simulink model "DAB_Converter_CPPS"  (R2025b)
settings: Solver=VariableStepAuto  StartTime=0.0  StopTime=inf  FixedStep=0.01  RelTol=1e-3
InitFcn:
  | % % 예시 코드 (SCPI 통신 객체가 obj_psu 라고 가정)
  | % % 시뮬레이션 시작 전에 미리 40V를 쏴줍니다.
  | % fprintf(obj_psu, 'VOLT 40');
  | % pause(0.5); % 장비가 인식할 시간 0.5초 대기
  | % disp('Initial Voltage Set to 40V');
undefined symbols (not defined in the file): dspblkCoreblockFVToolHelper, gcbh
libraries: instrumentseriallib x3, simulink x1, sldrtlib x1
settings Model: DataDictionary=DAB_Parameters.sldd  Creator=JWS  LastModifiedBy=pys30
settings DataIOCC: LimitDataPoints=on  MaxDataPoints=10000  SignalLogging=off  DSMLogging=off  ReturnWorkspaceOutputs=off

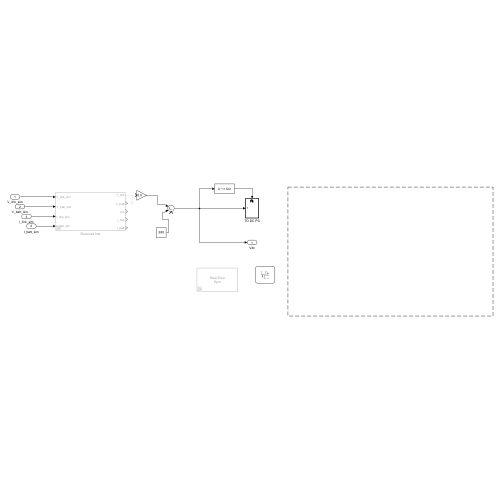
[thumbnail: Simulink's stored preview of the top-level diagram]
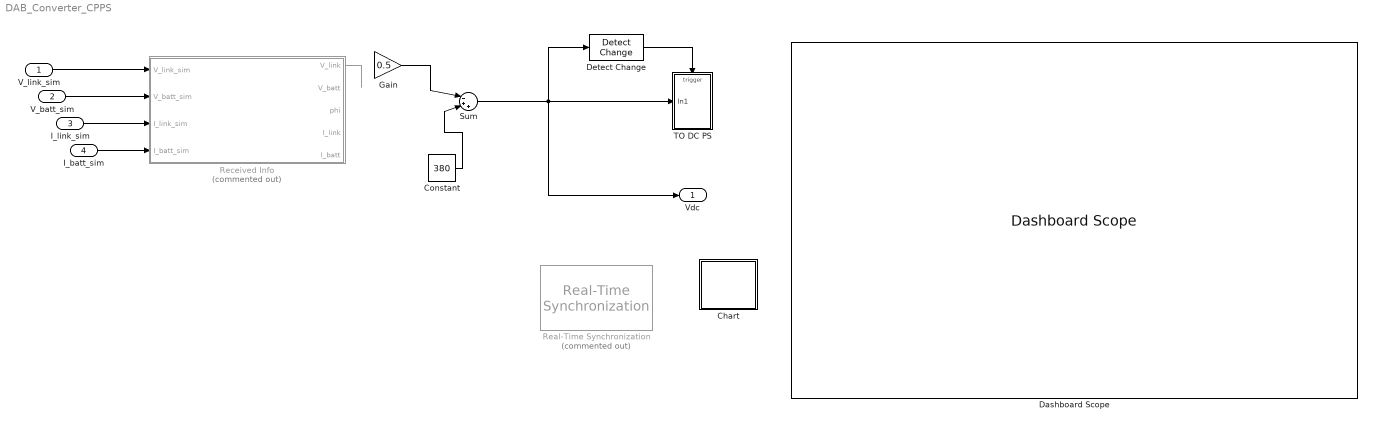
== system DAB_Converter_CPPS ==
  V_link_sim : Inport
  V_batt_sim : Inport  Port=2
  I_link_sim : Inport  Port=3
  I_batt_sim : Inport  Port=4
  Chart : Stateflow chart  TreatAsAtomicUnit=on
  Constant : Constant  Value=380
  Dashboard Scope : DashboardScope  FontColor=[0.0, 0.0, 0.0]
  Detect Change : simulink/Logic and Bit Operations/Detect Change  vinit=0  OutDataTypeStr=boolean
  Gain : Gain  Gain=0.5
  Real-Time Synchronization : sldrtlib/Real-Time Synchronization  Commented=on  SampleTime=0.01  MaxMissedTicks=inf  ShowMissedTicks=off  YieldWhenWaiting=off
  Received Info : Subsystem  Commented=on
  Sum : Sum  Inputs=|-++
  TO DC PS : Subsystem
  Vdc : Outport
  wires:
  Detect Change/1 -> TO DC PS/Trigger
  Constant/1 -> Sum/2
  Gain/1 -> Sum/1
  Sum/1 -> Vdc/1, Detect Change/1, TO DC PS/1(In1)
  Received Info/1(V_link) -> ?
  V_link_sim/1 -> Received Info/1(V_link_sim)
  V_batt_sim/1 -> Received Info/2(V_batt_sim)
  I_link_sim/1 -> Received Info/3(I_link_sim)
  I_batt_sim/1 -> Received Info/4(I_batt_sim)

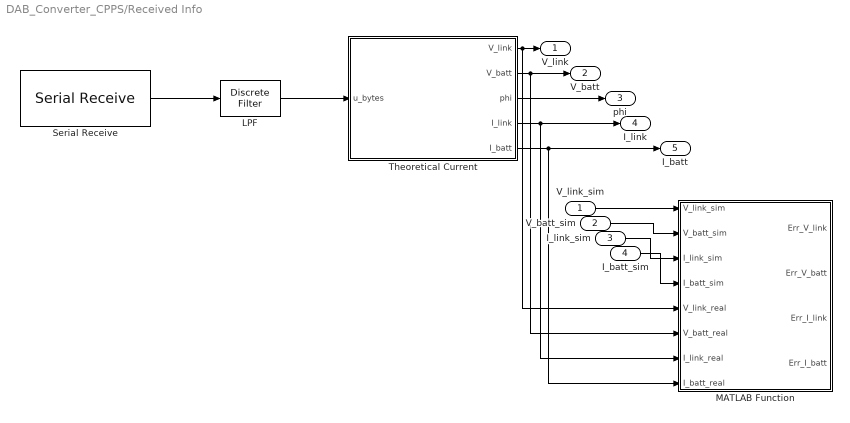
== system DAB_Converter_CPPS/Received Info ==
  V_link_sim : Inport
  V_batt_sim : Inport  Port=2
  I_link_sim : Inport  Port=3
  I_batt_sim : Inport  Port=4
  LPF : DiscreteFilter  LoadFcn=dspblkCoreblockFVToolHelper(gcbh,'load');
      settings: CopyFcn=dspblkCoreblockFVToolHelper(gcbh,'copy');  DeleteFcn=dspblkCoreblockFVToolHelper(gcbh,'close');  ModelCloseFcn=dspblkCoreblockFVToolHelper(gcbh,'close');  PreSaveFcn=dspblkCoreblockFVToolHelper(gcbh,'presave');  PostSaveFcn=dspblkCoreblockFVToolHelper(gcbh,'postsave');  CloseFcn=dspblkCoreblockFVToolHelper(gcbh,'close');
  MATLAB Function : MATLAB Function  TreatAsAtomicUnit=on
  Serial Receive : instrumentseriallib/Serial Receive  Priority=1  PortSel=COM5  Port=COM5  ComPort=COM5  DataType=uint8  SaveDataType=uint8  ToggleHeader=off  Header=[]  ToggleDataSize=on  DataSize=[1 1]  ToggleTerminator=off  Terminator=<none>  CustomTerminator=[]  InputFormat=Column major  EnableBlockingMode=on  ActionDataUnavailable=Output last received value  ActionWhenDataUnavailable=Output last received value  CustomValue=0  SampleTime=0.01  SimulateUsing=Interpreted execution  BlockInModel=on  aMode=1  LibraryInUse=instrumentlib
  Theoretical Current : MATLAB Function  TreatAsAtomicUnit=on
  V_link : Outport
  V_batt : Outport  Port=2
  phi : Outport  Port=3
  I_link : Outport  Port=4
  I_batt : Outport  Port=5
  wires:
  LPF/1 -> Theoretical Current/1(u_bytes)
  Serial Receive/1 -> LPF/1
  Theoretical Current/1(V_link) -> MATLAB Function/5(V_link_real), V_link/1
  Theoretical Current/2(V_batt) -> MATLAB Function/6(V_batt_real), V_batt/1
  Theoretical Current/3(phi) -> phi/1
  Theoretical Current/4(I_link) -> MATLAB Function/7(I_link_real), I_link/1
  Theoretical Current/5(I_batt) -> MATLAB Function/8(I_batt_real), I_batt/1
  I_batt_sim/1 -> MATLAB Function/4(I_batt_sim)
  I_link_sim/1 -> MATLAB Function/3(I_link_sim)
  V_batt_sim/1 -> MATLAB Function/2(V_batt_sim)
  V_link_sim/1 -> MATLAB Function/1(V_link_sim)

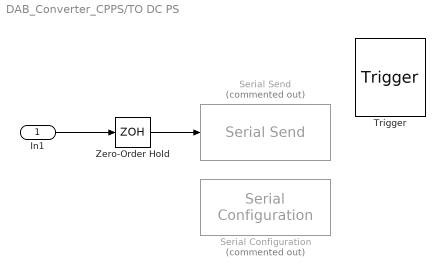
== system DAB_Converter_CPPS/TO DC PS ==
  In1 : Inport
  Trigger : TriggerPort  TriggerType=either  VariantControl=(inherit)  PortDimensions=1
  Serial Configuration : instrumentseriallib/Serial Configuration  Priority=-200000  Commented=on  PortSel=COM5  Port=COM5  ComPort=COM5  BaudRate=9600  DataBits=8  Parity=none  StopBits=1  ByteOrder=little-endian  FlowControl=none  Timeout=10  SimulateUsing=Interpreted execution  BlockInModel=on  aMode=1
  Serial Send : instrumentseriallib/Serial Send  Priority=1  Commented=on  PortSel=COM5  Port=COM5  ComPort=COM5  Header=[]  Terminator=<none>  CustomTerminator=[]  EnableBlockingMode=on  SimulateUsing=Interpreted execution  BlockInModel=on  aMode=1
  Zero-Order Hold : ZeroOrderHold  SampleTime=-1
  wires:
  In1/1 -> Zero-Order Hold/1
  Zero-Order Hold/1 -> Serial Send/1

== matlab function DAB_Converter_CPPS/Received Info/MATLAB Function ==
  data: V_link_sim input; Err_V_link output; V_batt_sim input; I_link_sim input; I_batt_sim input; V_link_real input; V_batt_real input; I_link_real input; I_batt_real input; Err_V_batt output; Err_I_link output; Err_I_batt output
function [Err_V_link, Err_V_batt, Err_I_link, Err_I_batt] = fcn_validator(V_link_sim, V_batt_sim, I_link_sim, I_batt_sim, V_link_real, V_batt_real, I_link_real, I_batt_real)
    % ---------------------------------------------------------------------
    % [2] 디지털 트윈 검증 (Digital Twin Validator)
    % ---------------------------------------------------------------------
    % 목적: 시뮬레이션(Sim) 결과와 실제(Real) 계측 값을 입력받아
    %       두 시스템 간의 오차(Error)를 실시간으로 계산함.
    %
    % 입력:
    %   - *_sim : 시뮬레이션 모델에서 계산된 전압/전류
    %   - *_real: 실제 하드웨어에서 계측 및 파싱된 전압/전류
    %
    % 출력:
    %   - Err_*: 오차 (실제값 - 시뮬레이션값)
    
    % 1. Link 전압 오차 (Real - Sim)
    Err_V_link = V_link_real - V_link_sim;
    
    % 2. Battery 전압 오차 (Real - Sim)
    Err_V_batt = V_batt_real - V_batt_sim;
    
    % 3. Link 전류 오차 (Real - Sim)
    Err_I_link = I_link_real - I_link_sim;
    
    % 4. Battery 전류 오차 (Real - Sim)
    Err_I_batt = I_batt_real - I_batt_sim;
    
    % [참고]
    % 오차가 (+)이면 실제값이 시뮬레이션보다 큰 상태
    % 오차가 (-)이면 실제값이 시뮬레이션보다 작은 상태
    % 오차가 0에 가까울수록 디지털 트윈의 정합성이 높음
end

== matlab function DAB_Converter_CPPS/Received Info/Theoretical Current ==
  data: u_bytes input; V_link output; V_batt output; phi output; I_link output; I_batt output
function [V_link, V_batt, phi, I_link, I_batt] = fcn_parser(u_bytes)
    % ---------------------------------------------------------------------
    % [1] 데이터 파싱 및 복구 (Data Parsing & Recovery)
    % ---------------------------------------------------------------------
    % 목적: MCU에서 보낸 문자열 패킷을 파싱하여 물리량으로 변환
    % 기능: 패킷 손실/깨짐 발생 시 직전 값을 유지(Hold)하여 시스템 안정성 확보
    
    % '이전 값'을 기억하기 위한 persistent 변수 선언
    persistent p_V_link p_V_batt p_phi p_I_link p_I_batt
    
    % 초기화 (시뮬레이션 첫 실행 시 기본값 설정)
    if isempty(p_V_link)
        p_V_link = 40; p_V_batt = 24; p_phi = 0;
        p_I_link = 0;  p_I_batt = 0;
    end
    
    % uint8 배열을 문자열로 변환 (C-String의 Null terminator 처리)
    str_data = char(u_bytes');
    null_idx = find(u_bytes == 0, 1);
    if ~isempty(null_idx)
        str_data = str_data(1:null_idx-1);
    end
    
    % 문자열을 숫자로 분해 (MCU 전송 포맷: "V1,V2,phi,I1,I2")
    values = sscanf(str_data, '%f,%f,%f,%f,%f');
    
    % 데이터 무결성 검사 (5개 데이터가 모두 정상 수신되었는지 확인)
    if length(values) == 5
        % 정상 수신 -> 현재 값 업데이트 및 '이전 값' 갱신
        V_link = values(1);
        V_batt = values(2);
        phi    = values(3);
        I_link = values(4);
        I_batt = values(5);
        
        % 다음 사이클을 위해 현재 값을 저장
        p_V_link = V_link; p_V_batt = V_batt; p_phi = phi;
        p_I_link = I_link; p_I_batt = I_batt;
    else
        % 수신 실패(데이터 깨짐 등) -> '이전 값' 유지 (Zero-Order Hold 효과)
        V_link = p_V_link;
        V_batt = p_V_batt;
        phi    = p_phi;
        I_link = p_I_link;
        I_batt = p_I_batt;
    end
end

== stateflow chart DAB_Converter_CPPS/Chart ==
